simulink model "GainCurveCLLCConverterReverse"  (R2026a)
settings: Solver=daessc  StopTime=0.5
PreLoadFcn:
  | if ~exist('CLLCDesign', 'var')
  | CLLCConverterDefaultInputParameters;
  | disp("default value loaded")
  | end
model workspace (MAT data in the model file):
  CLLCDesign.minGainFwd = simscape.Value
  CLLCDesign.minGainFwd.any = {0.75; '1'}
  CLLCDesign.maxGainFwd = simscape.Value
  CLLCDesign.maxGainFwd.any = {1.14285714286; '1'}
  CLLCDesign.avgGainFwd = simscape.Value
  CLLCDesign.avgGainFwd.any = {0.933333333333; '1'}
  CLLCDesign.maxGainRev = simscape.Value
  CLLCDesign.maxGainRev.any = {1.33333333333; '1'}
  CLLCDesign.minGainRev = simscape.Value
  CLLCDesign.minGainRev.any = {0.875; '1'}
  CLLCDesign.avgGainRev = simscape.Value
  CLLCDesign.avgGainRev.any = {1.07142857143; '1'}
  CLLCDesign.deadTime = 2e-07
  CLLCDesign.Co = 0.00122448979592
  CLLCDesign.C1 = 5.58505360638e-07
  CLLCDesign.L1 = 4.53537202967e-06
  CLLCDesign.C2 = 6.47552771454e-07
  CLLCDesign.L2 = 3.91130483839e-06
  CLLCDesign.Lm = 2.7212232178e-05
  CLLCDesign.N2 = 10
  CLLCDesign.N1 = 11
  CLLCDesign.turnsRatio = 1.1
  CLLCDesign.resonantFreq = 100000
  CLLCDesign.Cparasitic = 2e-10
  CLLCDesign.Llk1 = 4.53537202967e-06
  CLLCDesign.Llk2 = 3.91130483839e-06
  CLLCDesign.Rco = 0.02
  CLLCDesign.R1 = 0.0001
  CLLCDesign.R2 = 0.0001
  CLLCDesign.Rcr1 = 0.0001
  CLLCDesign.Rcr2 = 0.0001
  LLCDesign.minGain = simscape.Value
  LLCDesign.minGain.any = {0.75; '1'}
  LLCDesign.maxGain = simscape.Value
  LLCDesign.maxGain.any = {1.14285714286; '1'}
  LLCDesign.avgGain = simscape.Value
  LLCDesign.avgGain.any = {0.933333333333; '1'}
  LLCDesign.deadTime = 2.5e-07
  LLCDesign.Co = 0.000816326530612
  LLCDesign.C = 2.32710566933e-07
  LLCDesign.L = 1.08848928712e-05
  LLCDesign.Lm = 4.35395714848e-05
  LLCDesign.N2 = 10
  LLCDesign.N1 = 11
  LLCDesign.resonantFreq = 100000
  LLCDesign.Cparasitic = 2e-10
  LLCDesign.Llk1 = 1.03406482276e-05
  LLCDesign.Llk2 = 4.4978896162e-07
  LLCDesign.Rco = 0.02
  LLCDesign.R1 = 0.0001
  LLCDesign.R2 = 0.0001
  LLCDesign.Rcr = 0.0001
libraries: fl_lib x9, nesl_utility x4, ee_lib x1
settings Model: Creator=vsolaise  LastModifiedBy=vsolaise
settings SimscapeCC: SimscapeNominalValues="[{\"value\":\"1\",\"unit\":\"A\"},{\"value\":\"1\",\"unit\":\"bar\"},{\"value\":\"1\",\"unit\":\"cm^2\"},{\"value\":\"1\",\"unit\":\"cm^3/s\"},{\"value\":\"1\",\"unit\":\"kJ/kg\"},{\"value\":\"1\",\"unit\":\"kW\"},{\"value\":\"1\",\"unit\":\"l\"},{\"value\":\"1\",\"unit\":\"N\"},{\"value\":\"1\",\"unit\":\"N*m\"},{\"value\":\"1\",\"unit\":\"V\"}]"  SimscapeLogType=none  SimscapeLogDataHistory=5000.0

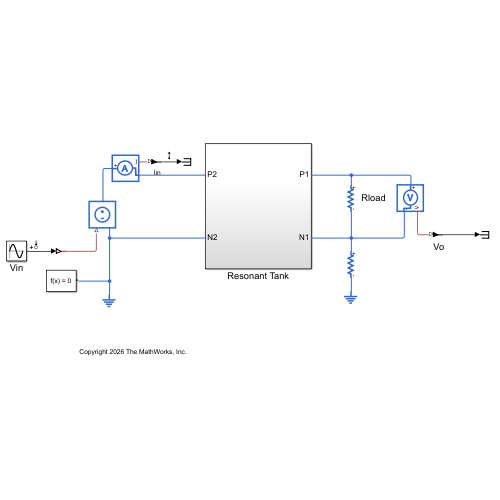
[thumbnail: Simulink's stored preview of the top-level diagram]
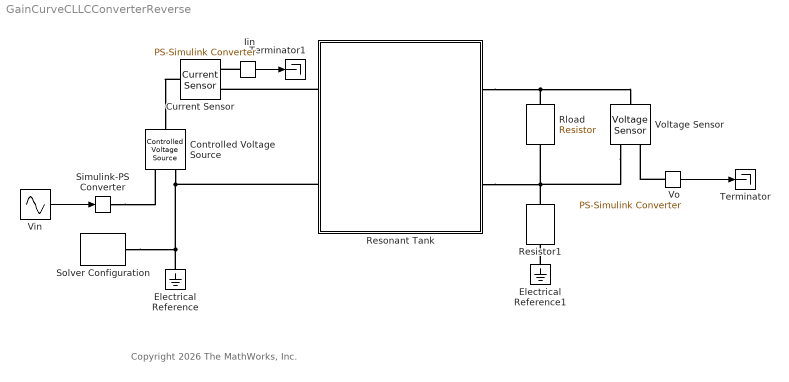
== system GainCurveCLLCConverterReverse ==
  note: Copyright 2026 The MathWorks, Inc.
  Controlled Voltage Source : fl_lib/Electrical/Electrical Sources/Controlled Voltage Source
  Current Sensor : fl_lib/Electrical/Electrical Sensors/Current Sensor
  Electrical Reference : fl_lib/Electrical/Electrical Elements/Electrical Reference
  Electrical Reference1 : fl_lib/Electrical/Electrical Elements/Electrical Reference
  Iin : nesl_utility/PS-Simulink Converter  PhysicalDomain=network_engine_domain  SubClassName=ps_output  LeftPortType=input  RightPortType=output  PseudoPeriodic=off  Frequencies=[]  VectorFormat=inherit  Unit=inherit  AffineConversion=off
  Resistor1 : fl_lib/Electrical/Electrical Elements/Resistor  R=1e6 Ohm  i_specify=off  i_priority=None  i=0 A  i_nominal_specify=off  i_nominal_value=1  i_nominal_unit=A  v_specify=off  v_priority=None  v=0 V  v_nominal_specify=off  v_nominal_value=1  v_nominal_unit=V
  Resonant Tank : Subsystem
  Rload : fl_lib/Electrical/Electrical Elements/Resistor  R=8.2062 Ohm  i_specify=off  i_priority=None  i=0 A  i_nominal_specify=off  i_nominal_value=1  i_nominal_unit=A  v_specify=off  v_priority=None  v=0 V  v_nominal_specify=off  v_nominal_value=1  v_nominal_unit=V
  Simulink-PS Converter : nesl_utility/Simulink-PS Converter  PhysicalDomain=network_engine_domain  SubClassName=ps_input  LeftPortType=input  RightPortType=output  PseudoPeriodic=off  Frequencies=[]  NoiseDistribution=none  NoiseParameters=[]  Unit=1  AffineConversion=off  FilteringAndDerivatives=zero  SimscapeFilterOrder=1  InputFilterTimeConstant=0.001  UdotUserProvided=0
  Solver Configuration : nesl_utility/Solver Configuration  PhysicalDomain=network_engine_domain  SubClassName=solver  LeftPortType=input  RightPortType=generic  Tones=[]  Harmonics=[]  SimulateNoise=off  Profile=off  UseLocalSampling=off  EnableSwitchedLinearOptims=on  FrequencyDomain=off  UseCCode=off  RelTol=0.001  AbsTol=0.001  MinStep=1e-09  ToWorkspace=off  RevertToSquareIcSolve=off  NumHomotopyIterations=100  PhasorMode=off  PhasorModeNumHarmonics=1  ConsistencySolver=NEWTON_XTOL_AFTER_FTOL  CanonicalOrdering=UNORDERED  OptimizeIntermediates=UNOPTIMIZED  IndexReductionMethod=DerivativeReplacement  DoDC=off  ResidualTolerance=1e-09  ConsistencyTolSource=GLOBAL  ConsistencyAbsTol=0.001  ConsistencyRelTol=0.001  ConsistencyTolFactor=0.001  UseLocalSolver=off  LocalSolverChoice=NE_BACKWARD_EULER_ADVANCER  ResolveIndetEquations=on  FunctionEvalNumThread=1  LocalSolverSampleTime=0.001  DoFixedCost=off  MaxNonlinIter=3  MaxModeIter=2  ComputeImpulses=off  ImpulseIterations=2  LinearAlgebra=auto  LinearAlgebraNumThread=0  EquationFormulation=NE_TIME_EF  DelaysMemoryBudget=1024  AutomaticFiltering=on  FilteringTimeConstant=0.001  PartitionStorageMethod=AS_NEEDED  PartitionMemoryBudget=1024  PartitionMethod=ROBUST  MultibodyUseLocalSolver=off  MultibodyLocalSolverChoice=ODE1  MultibodyLocalSolverSampleTime=0.001
  Terminator : Terminator
  Terminator1 : Terminator
  Vin : Sin  SampleTime=0
  Vo : nesl_utility/PS-Simulink Converter  PhysicalDomain=network_engine_domain  SubClassName=ps_output  LeftPortType=input  RightPortType=output  PseudoPeriodic=off  Frequencies=[]  VectorFormat=inherit  Unit=inherit  AffineConversion=off
  Voltage Sensor : fl_lib/Electrical/Electrical Sensors/Voltage Sensor
  wires:
  Vo/1 -> Terminator/1
  Vin/1 -> Simulink-PS Converter/1
  Iin/1 -> Terminator1/1
  connections:
  Simulink-PS Converter/RConn1 -- Controlled Voltage Source/RConn1
  Rload/LConn1 -- Resonant Tank/LConn1 -- Voltage Sensor/LConn1
  Vo/LConn1 -- Voltage Sensor/RConn1
  Electrical Reference1/LConn1 -- Resistor1/RConn1
  Electrical Reference/LConn1 -- Solver Configuration/RConn1 -- Resonant Tank/RConn2 -- Controlled Voltage Source/RConn2
  Voltage Sensor/RConn2 -- Rload/RConn1 -- Resonant Tank/LConn2 -- Resistor1/LConn1
  Resonant Tank/RConn1 -- Current Sensor/RConn2
  Current Sensor/LConn1 -- Controlled Voltage Source/LConn1
  Iin/LConn1 -- Current Sensor/RConn1

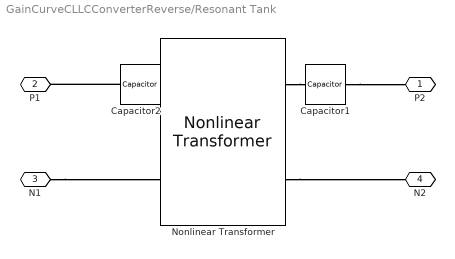
== system GainCurveCLLCConverterReverse/Resonant Tank ==
  Capacitor1 : fl_lib/Electrical/Electrical Elements/Capacitor  c=CLLCDesign.C2 F  r=CLLCDesign.Rcr2 Ohm  g=0 1/Ohm  i_specify=off  i_priority=None  i=0 A  i_nominal_specify=off  i_nominal_value=1  i_nominal_unit=A  v_specify=off  v_priority=None  v=0 V  v_nominal_specify=off  v_nominal_value=1  v_nominal_unit=V  vc_specify=off  vc_priority=High  vc=0 V  vc_nominal_specify=off  vc_nominal_value=1  vc_nominal_unit=V
  Capacitor2 : fl_lib/Electrical/Electrical Elements/Capacitor  c=CLLCDesign.C1 F  r=CLLCDesign.Rcr1 Ohm  g=0 1/Ohm  i_specify=off  i_priority=None  i=0 A  i_nominal_specify=off  i_nominal_value=1  i_nominal_unit=A  v_specify=off  v_priority=None  v=0 V  v_nominal_specify=off  v_nominal_value=1  v_nominal_unit=V  vc_specify=off  vc_priority=High  vc=0 V  vc_nominal_specify=off  vc_nominal_value=1  vc_nominal_unit=V
  Nonlinear Transformer : ee_lib/Passive/Transformers/Nonlinear Transformer  Nw=CLLCDesign.N1  Nw2=CLLCDesign.N2  winding_param_option=2  Req=0.01 Ohm  Leq=0.0001 H  R_1=CLLCDesign.R1 Ohm  L_1=CLLCDesign.Llk1 H  R_2=CLLCDesign.R2 Ohm  L_2=CLLCDesign.Llk2 H  averaging_period=0 s  R_m=5000 Ohm  parameterization_option=1  H_data=[0, 200, 400, 600, 800, 1000] A/m  B_data=[0, .81, 1.25, 1.42, 1.48, 1.49] T  length_effective=0.2 m  area_effective=2e-4 m^2  L=CLLCDesign.Lm H  L_sat=1e-2 H  current_data=[0, .4, .8, 1.2, 1.6, 2] A  magnetic_flux_data=[0, .161, .25, .284, .295, .299] .* 1e-3 Wb  magnetic_flux_sat=1.6e-04 Wb  dBdH0=0.005 T*m/A  B1=1.49 T  H1=1000 A/m  c=0.1  K=200 A/m  alpha=1e-4  interpolation_option=1  Leq_i0=0 A  L1_i0=0 A  L2_i0=0 A  x0_option=1  i_L0=0 A  phi0=0 Wb  B0=0 T  H0=0 A/m  Leq_g=1e-9 1/Ohm  L1_g=1e-9 1/Ohm  L2_g=1e-9 1/Ohm
  P2 : PMIOPort  Side=Right
  P1 : PMIOPort  Port=2  Side=Left
  N1 : PMIOPort  Port=3  Side=Left
  N2 : PMIOPort  Port=4  Side=Right
  connections:
  Nonlinear Transformer/LConn1 -- Capacitor2/RConn1
  Nonlinear Transformer/RConn1 -- Capacitor1/LConn1
  N1/RConn1 -- Nonlinear Transformer/LConn2
  Capacitor2/LConn1 -- P1/RConn1
  Nonlinear Transformer/RConn2 -- N2/RConn1
  Capacitor1/RConn1 -- P2/RConn1
